simulink model "part1-2"  (R2018b)
settings: Solver=VariableStepAuto  StartTime=0.0  StopTime=200  RelTol=1e-3
settings Model: Creator=Engineer  LastModifiedBy=Engineer

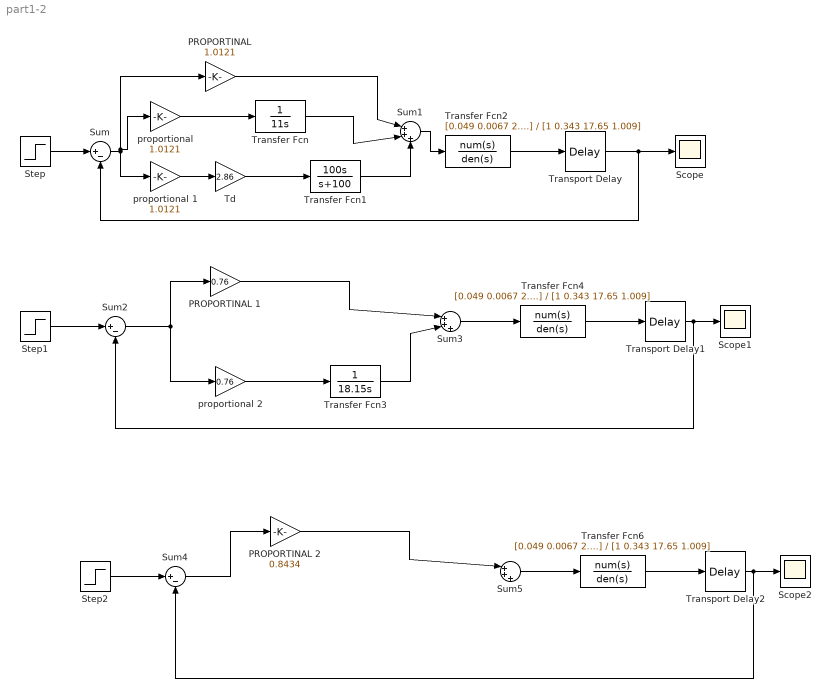
== system part1-2 ==
  "PROPORTINAL " : Gain  Gain=1.0121
  PROPORTINAL 1 : Gain  Gain=0.76
  PROPORTINAL 2 : Gain  Gain=0.8434
  Scope : Scope
  Scope1 : Scope
  Scope2 : Scope
  Step : Step  Time=0  SampleTime=0
  Step1 : Step  Time=0  SampleTime=0
  Step2 : Step  Time=0  SampleTime=0
  Sum : Sum  Inputs=|+-
  Sum1 : Sum  Inputs=|+++
  Sum2 : Sum  Inputs=|+-
  Sum3 : Sum  Inputs=|+++
  Sum4 : Sum  Inputs=|+-
  Sum5 : Sum  Inputs=|+++
  Td : Gain  Gain=2.86
  Transfer Fcn : TransferFcn  Denominator=[11 0]
  Transfer Fcn1 : TransferFcn  Numerator=[100 0]  Denominator=[1 100]
  Transfer Fcn2 : TransferFcn  Numerator=[0.049 0.0067 2.991]  Denominator=[1 0.343 17.65 1.009]
  Transfer Fcn3 : TransferFcn  Denominator=[18.15 0]
  Transfer Fcn4 : TransferFcn  Numerator=[0.049 0.0067 2.991]  Denominator=[1 0.343 17.65 1.009]
  Transfer Fcn6 : TransferFcn  Numerator=[0.049 0.0067 2.991]  Denominator=[1 0.343 17.65 1.009]
  Transport Delay : TransportDelay  DelayTime=5
  Transport Delay1 : TransportDelay  DelayTime=5
  Transport Delay2 : TransportDelay  DelayTime=5
  "proportional " : Gain  Gain=1.0121
  proportional 1 : Gain  Gain=1.0121
  proportional 2 : Gain  Gain=0.76
  wires:
  Step/1 -> Sum/1
  Transfer Fcn2/1 -> Transport Delay/1
  Transport Delay/1 -> Sum/2, Scope/1
  Sum/1 -> "PROPORTINAL "/1, "proportional "/1, proportional 1/1
  "proportional "/1 -> Transfer Fcn/1
  Td/1 -> Transfer Fcn1/1
  "PROPORTINAL "/1 -> Sum1/1
  Sum1/1 -> Transfer Fcn2/1
  Transfer Fcn/1 -> Sum1/2
  Transfer Fcn1/1 -> Sum1/3
  proportional 1/1 -> Td/1
  Step1/1 -> Sum2/1
  proportional 2/1 -> Transfer Fcn3/1
  Sum2/1 -> PROPORTINAL 1/1, proportional 2/1
  PROPORTINAL 1/1 -> Sum3/1
  Transfer Fcn3/1 -> Sum3/2
  Sum3/1 -> Transfer Fcn4/1
  Transfer Fcn4/1 -> Transport Delay1/1
  Transport Delay1/1 -> Sum2/2, Scope1/1
  Transport Delay2/1 -> Sum4/2, Scope2/1
  Sum4/1 -> PROPORTINAL 2/1
  Sum5/1 -> Transfer Fcn6/1
  Transfer Fcn6/1 -> Transport Delay2/1
  PROPORTINAL 2/1 -> Sum5/1
  Step2/1 -> Sum4/1
